simulink model "OBC"  (R2023a)
settings: Solver=VariableStepAuto  StartTime=0.0  StopTime=10.0  RelTol=1e-3
libraries: simulink x5
settings Model: DataDictionary=SatelliteTelescope.sldd  Creator=Ren4  LastModifiedBy=Ren4

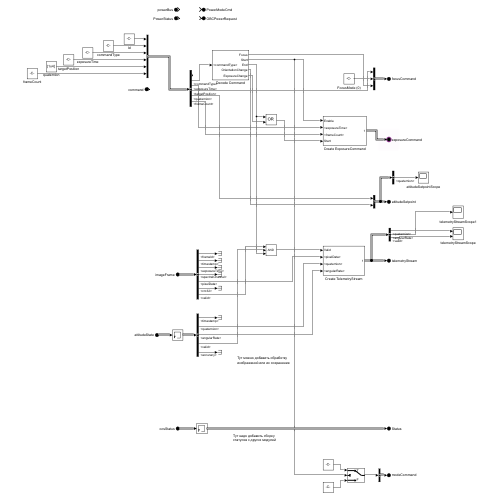
[thumbnail: Simulink's stored preview of the top-level diagram]
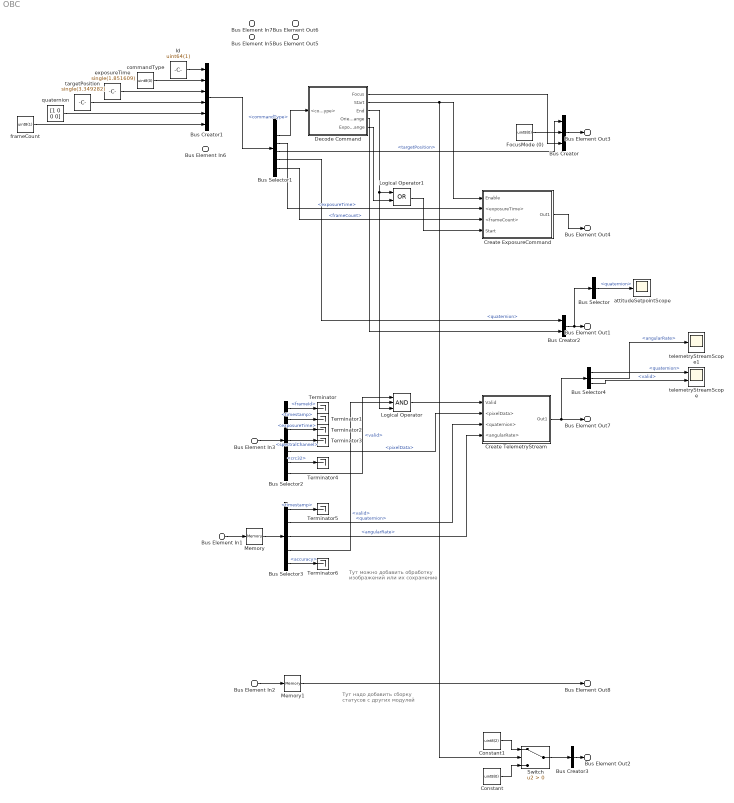
== system OBC ==
  note: Тут надо добавить сборку
      | статусов с других модулей
  note: Тут можно добавить обработку
      | изображений или их сохранение
  Bus Element In7 : Inport  PortName=powerBus
  Bus Element In6 : Inport  Port=2  PortName=command
  Bus Element In5 : Inport  Port=3  PortName=PowerStatus
  Bus Element In3 : Inport  Port=4  PortName=imageFrame
  Bus Element In1 : Inport  Port=5  PortName=attitudeState
  Bus Element In2 : Inport  Port=6  PortName=ocsStatus
  Bus Creator : BusCreator  Inputs=3  OutDataTypeStr=Bus: FocusCommand_IF
      settings: InheritFromInputs=off
  Bus Creator1 : BusCreator  Inputs=6  OutDataTypeStr=Bus: Command_IF
      settings: InheritFromInputs=off
  Bus Creator2 : BusCreator  Inputs=2  OutDataTypeStr=Bus: AttitudeSetpoint_IF
      settings: InheritFromInputs=off
  Bus Creator3 : BusCreator  Inputs=1  OutDataTypeStr=Bus: ModeCommand_IF
      settings: InheritFromInputs=off
  Bus Selector : BusSelector  OutputSignals=quaternion
  Bus Selector1 : BusSelector  OutputSignals=comamndId,commandType,exposureTime,targetPosition,quaternion,frameCount
  Bus Selector2 : BusSelector  OutputSignals=frameId,timestamp,exposureTime,spectralChannel,pixelData,crc32,valid
  Bus Selector3 : BusSelector  OutputSignals=timestamp,quaternion,angularRate,valid,accuracy
  Bus Selector4 : BusSelector  OutputSignals=quaternion,angularRate,valid
  Constant : Constant  Value=uint8(0)
  Constant1 : Constant  Value=uint8(2)
  Create ExposureCommand : Subsystem
  Create TelemetryStream : Subsystem
  Decode Command : Subsystem
  FocusMode (0) : Constant  Value=uint8(0)
  Id : Constant  Value=uint64(1)
  Logical Operator : Logic  Inputs=3  AllPortsSameDT=off  OutDataTypeStr=boolean
  Logical Operator1 : Logic  Operator=OR  AllPortsSameDT=off  OutDataTypeStr=boolean
  Memory : Memory
  Memory1 : Memory
  Switch : Switch  Criteria=u2 > Threshold  SaturateOnIntegerOverflow=off  InputSameDT=off
  Terminator{,1..6} (7 alike) : Terminator
  attitudeSetpointScope : Scope
  commandType : Constant  Value=uint8(0)
  exposureTime : Constant  Value=single(1.851609)
  frameCount : Constant  Value=uint8(1)
  quaternion : Constant  Value=[1 0 0 0]
  targetPosition : Constant  Value=single(3.349282)
  telemetryStreamScope : Scope  NumInputPorts=2
  telemetryStreamScope1 : Scope
  Bus Element Out5 : Outport  PortName=OBCPowerRequest
  Bus Element Out2 : Outport  Port=2  PortName=modeCommand
  Bus Element Out6 : Outport  Port=3  PortName=PowerModeCmd
  Bus Element Out8 : Outport  Port=4  PortName=Status
  Bus Element Out7 : Outport  Port=5  PortName=telemetryStream
  Bus Element Out3 : Outport  Port=6  PortName=focusCommand
  Bus Element Out4 : Outport  Port=7  PortName=exposureCommand
  Bus Element Out1 : Outport  Port=8  PortName=attitudeSetpoint
  wires:
  Bus Creator/1 -> Bus Element Out3/1
  FocusMode (0)/1 -> Bus Creator/2
  Bus Selector1/4 -> Bus Creator/1  "<targetPosition>"
  Bus Creator2/1 -> Bus Selector/1, Bus Element Out1/1
  Bus Selector1/5 -> Bus Creator2/1  "<quaternion>"
  Bus Element In3/1 -> Bus Selector2/1
  Bus Element In1/1 -> Memory/1
  Bus Selector2/7 -> Logical Operator/1  "<valid>"
  Bus Selector3/4 -> Logical Operator/2  "<valid>"
  Decode Command/3(End) -> Logical Operator/3, Logical Operator1/1
  Bus Selector1/2 -> Decode Command/1(<commandType>)  "<commandType>"
  Decode Command/1(Focus) -> Bus Creator/3
  Bus Selector2/1 -> Terminator/1  "<frameId>"
  Bus Selector2/2 -> Terminator1/1  "<timestamp>"
  Bus Selector2/3 -> Terminator2/1  "<exposureTime>"
  Bus Selector2/4 -> Terminator3/1  "<spectralChannel>"
  Bus Selector2/6 -> Terminator4/1  "<crc32>"
  Bus Selector3/1 -> Terminator5/1  "<timestamp>"
  Bus Selector3/5 -> Terminator6/1  "<accuracy>"
  Decode Command/4(OrientationChange) -> Bus Creator2/2
  Bus Element In2/1 -> Memory1/1
  Decode Command/5(ExposureChange) -> Logical Operator1/2
  Memory/1 -> Bus Selector3/1
  Decode Command/2(Start) -> Create ExposureCommand/1(Enable), Switch/2
  Bus Selector1/3 -> Create ExposureCommand/2(<exposureTime>)  "<exposureTime>"
  Bus Selector1/6 -> Create ExposureCommand/3(<frameCount>)  "<frameCount>"
  Logical Operator1/1 -> Create ExposureCommand/4(Start)
  Create ExposureCommand/1(Out1) -> Bus Element Out4/1
  Logical Operator/1 -> Create TelemetryStream/1(Valid)
  Bus Selector2/5 -> Create TelemetryStream/2(<pixelData>)  "<pixelData>"
  Bus Selector3/2 -> Create TelemetryStream/3(<quaternion>)  "<quaternion>"
  Bus Selector3/3 -> Create TelemetryStream/4(<angularRate>)  "<angularRate>"
  Create TelemetryStream/1(Out1) -> Bus Selector4/1, Bus Element Out7/1
  Constant/1 -> Switch/3
  Constant1/1 -> Switch/1
  Bus Creator1/1 -> Bus Selector1/1
  Id/1 -> Bus Creator1/1
  commandType/1 -> Bus Creator1/2
  exposureTime/1 -> Bus Creator1/3
  targetPosition/1 -> Bus Creator1/4
  quaternion/1 -> Bus Creator1/5
  frameCount/1 -> Bus Creator1/6
  Switch/1 -> Bus Creator3/1
  Bus Creator3/1 -> Bus Element Out2/1
  Memory1/1 -> Bus Element Out8/1
  Bus Selector/1 -> attitudeSetpointScope/1  "<quaternion>"
  Bus Selector4/1 -> telemetryStreamScope/1  "<quaternion>"
  Bus Selector4/3 -> telemetryStreamScope/2  "<valid>"
  Bus Selector4/2 -> telemetryStreamScope1/1  "<angularRate>"

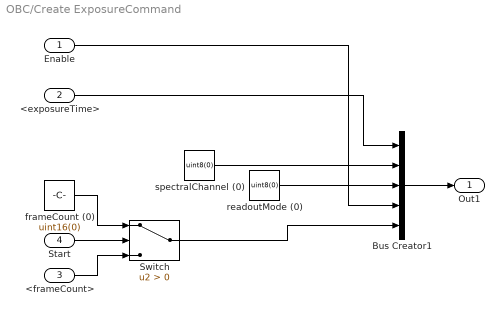
== system OBC/Create ExposureCommand ==
  Enable : Inport
  <exposureTime> : Inport  Port=2
  <frameCount> : Inport  Port=3
  Start : Inport  Port=4
  Bus Creator1 : BusCreator  Inputs=5  OutDataTypeStr=Bus: ExposureCommand_IF
      settings: InheritFromInputs=off
  Switch : Switch  Criteria=u2 > Threshold  SaturateOnIntegerOverflow=off  InputSameDT=off
  frameCount (0) : Constant  Value=uint16(0)
  readoutMode (0) : Constant  Value=uint8(0)
  spectralChannel (0) : Constant  Value=uint8(0)
  Out1 : Outport
  wires:
  spectralChannel (0)/1 -> Bus Creator1/2
  readoutMode (0)/1 -> Bus Creator1/3
  <frameCount>/1 -> Switch/3
  Bus Creator1/1 -> Out1/1
  frameCount (0)/1 -> Switch/1
  Enable/1 -> Bus Creator1/4
  Start/1 -> Switch/2
  Switch/1 -> Bus Creator1/5
  <exposureTime>/1 -> Bus Creator1/1

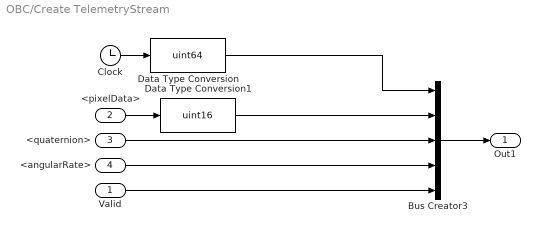
== system OBC/Create TelemetryStream ==
  Valid : Inport
  <pixelData> : Inport  Port=2
  <quaternion> : Inport  Port=3
  <angularRate> : Inport  Port=4
  Bus Creator3 : BusCreator  Inputs=5  OutDataTypeStr=Bus: TelemetryStream_IF
      settings: InheritFromInputs=off
  Clock : Clock
  Data Type Conversion : DataTypeConversion  OutDataTypeStr=uint64  SaturateOnIntegerOverflow=off  RndMeth=Floor
  Data Type Conversion1 : DataTypeConversion  OutDataTypeStr=uint16  SaturateOnIntegerOverflow=off  RndMeth=Floor
  Out1 : Outport
  wires:
  Data Type Conversion1/1 -> Bus Creator3/2
  Clock/1 -> Data Type Conversion/1
  <pixelData>/1 -> Data Type Conversion1/1
  Data Type Conversion/1 -> Bus Creator3/1
  Valid/1 -> Bus Creator3/5
  <angularRate>/1 -> Bus Creator3/4
  <quaternion>/1 -> Bus Creator3/3
  Bus Creator3/1 -> Out1/1

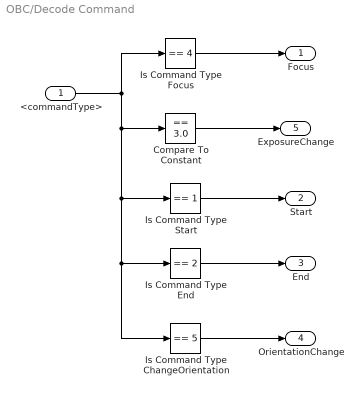
== system OBC/Decode Command ==
  <commandType> : Inport
  Compare To Constant : simulink/Logic and Bit Operations/Compare To Constant  relop===  const=3.0  OutDataTypeStr=boolean
  Is Command Type ChangeOrientation : simulink/Logic and Bit Operations/Compare To Constant  relop===  const=5  OutDataTypeStr=boolean
  Is Command Type End : simulink/Logic and Bit Operations/Compare To Constant  relop===  const=2  OutDataTypeStr=boolean
  Is Command Type Focus : simulink/Logic and Bit Operations/Compare To Constant  relop===  const=4  OutDataTypeStr=boolean
  Is Command Type Start : simulink/Logic and Bit Operations/Compare To Constant  relop===  const=1  OutDataTypeStr=boolean
  Focus : Outport
  Start : Outport  Port=2
  End : Outport  Port=3
  OrientationChange : Outport  Port=4
  ExposureChange : Outport  Port=5
  wires:
  Is Command Type Focus/1 -> Focus/1
  <commandType>/1 -> Is Command Type ChangeOrientation/1, Is Command Type End/1, Is Command Type Start/1, Compare To Constant/1, Is Command Type Focus/1
  Is Command Type End/1 -> End/1
  Is Command Type Start/1 -> Start/1
  Is Command Type ChangeOrientation/1 -> OrientationChange/1
  Compare To Constant/1 -> ExposureChange/1
